simulink model "cp6_ej3"  (R2026a)
settings: Solver=VariableStepAuto  StopTime=30  MaxStep=0.01
settings Model: Creator=benja  LastModifiedBy=benja

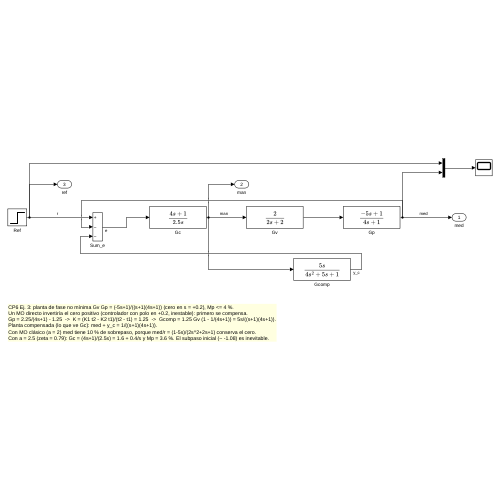
[thumbnail: Simulink's stored preview of the top-level diagram]
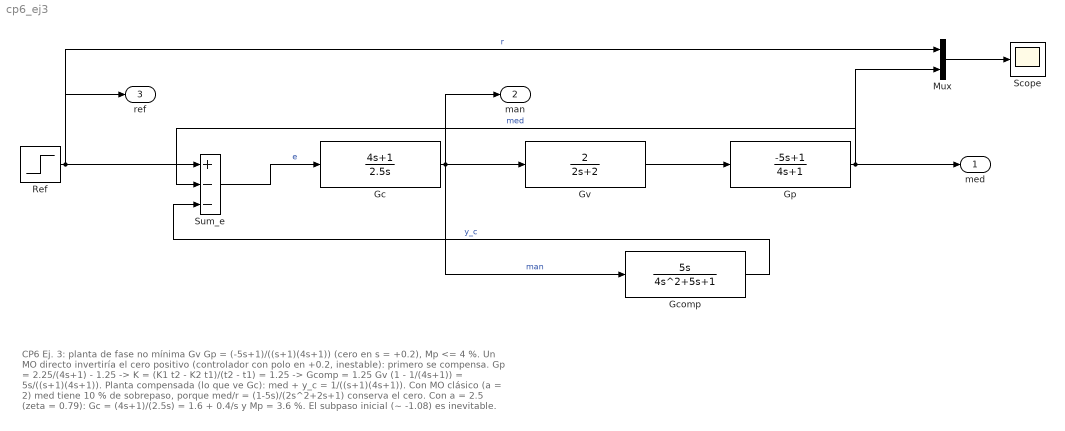
== system cp6_ej3 ==
  note: CP6 Ej. 3: planta de fase no mínima Gv Gp = (-5s+1)/((s+1)(4s+1)) (cero en s = +0.2), Mp <= 4 %.
      | Un MO directo invertiría el cero positivo (controlador con polo en +0.2, inestable): primero se compensa.
      | Gp = 2.25/(4s+1) - 1.25  ->  K = (K1 t2 - K2 t1)/(t2 - t1) = 1.25  ->  Gcomp = 1.25 Gv (1 - 1/(4s+1)) = 5s/((s+1)(4s+1)).
      | Planta compensada (lo que ve Gc): med + y_c = 1/((s+1)(4s+1)).
      | Con MO clásico (a = 2) med tiene 10 % de sobrepaso, porque med/r = (1-5s)/(2s^2+2s+1) conserva el cero.
      | Con a = 2.5 (zeta = 0.79): Gc = (4s+1)/(2.5s) = 1.6 + 0.4/s y Mp = 3.6 %. El subpaso inicial (~ -1.08) es inevitable.
  Gc : TransferFcn  Numerator=[4 1]  Denominator=[2.5 0]
  Gcomp : TransferFcn  Numerator=[5 0]  Denominator=[4 5 1]
  Gp : TransferFcn  Numerator=[-5 1]  Denominator=[4 1]
  Gv : TransferFcn  Numerator=2  Denominator=[2 2]
  Mux : Mux  Inputs=2
  Ref : Step  SampleTime=0
  Scope : Scope
  Sum_e : Sum  Inputs=+--
  med : Outport
  man : Outport  Port=2
  ref : Outport  Port=3
  wires:
  Ref/1 -> Sum_e/1, ref/1, Mux/1  "r"
  Sum_e/1 -> Gc/1  "e"
  Gc/1 -> Gv/1, Gcomp/1, man/1  "man"
  Gv/1 -> Gp/1
  Gp/1 -> med/1, Sum_e/2, Mux/2  "med"
  Gcomp/1 -> Sum_e/3  "y_c"
  Mux/1 -> Scope/1
